simulink model "etudeinfluenceamortissementc"  (R2024a)
settings: Solver=VariableStepAuto  StartTime=0.0  StopTime=2  RelTol=1e-3
values from neighbouring files (symbols this model uses):
  c_list = [750, 1500, 2250]    [etude_influence_amortissement_c.m]
  k = 20000    [air_gear.m]    (also in etude_influence_amortissement_c.m; etude_influence_raideur_k.m = k_list(i))
  m = 100    [air_gear.m]    (also in etude_influence_amortissement_c.m; etude_influence_raideur_k.m)
settings Model: Creator=nnguy  LastModifiedBy=nnguy

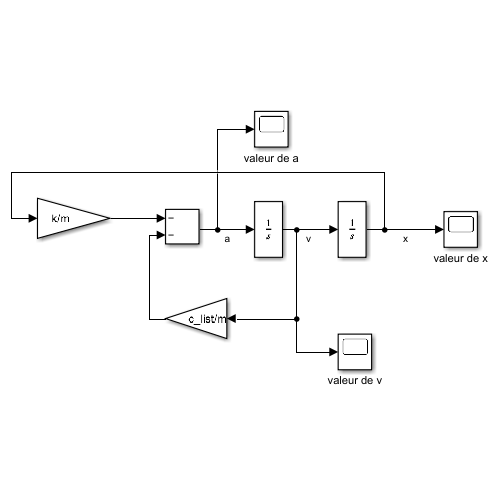
[thumbnail: Simulink's stored preview of the top-level diagram]
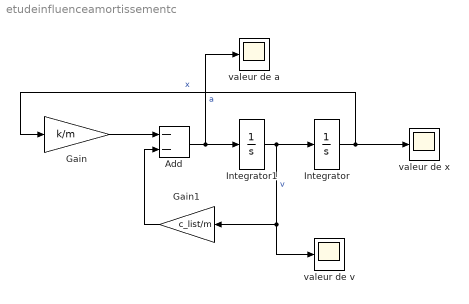
== system etudeinfluenceamortissementc ==
  Add : Sum  Inputs=--
  Gain : Gain  Gain=k/m
  Gain1 : Gain  Gain=c_list/m
  Integrator : Integrator
  Integrator1 : Integrator  InitialCondition=1
  valeur de a : Scope
  valeur de v : Scope
  valeur de x : Scope
  wires:
  Add/1 -> valeur de a/1, Integrator1/1  "a"
  Integrator/1 -> Gain/1, valeur de x/1  "x"
  Integrator1/1 -> valeur de v/1, Gain1/1, Integrator/1  "v"
  Gain1/1 -> Add/2
  Gain/1 -> Add/1
